simulink model "sf_debouncer_using_duration"  (R2025b)
settings: Solver=VariableStepDiscrete  StartTime=0.0  StopTime=6  RelTol=1e-3  EnableMultiTasking=on
settings Model: Creator=The MathWorks, Inc.  LastModifiedBy=The MathWorks, Inc.
settings SolverCC: AlgebraicLoopSolver=TrustRegion  InsertRTBMode=Auto
settings DataIOCC: LimitDataPoints=on  SaveFormat=Array  ReturnWorkspaceOutputs=off
settings OptimizationCC: ReuseModelBlockBuffer=off  ExpressionDepthLimit=2147483647.0  InitFltsAndDblsToZero=on  EfficientMapNaN2IntZero=off  LifeSpan=inf
settings DebuggingCC: SaveWithParameterizedLinksMsg=none  UnderspecifiedInitializationDetection=Classic  MergeDetectMultiDrivingBlocksExec=none  SignalResolutionControl=TryResolveAllWithWarning  SolverPrmCheckMsg=warning  MultiTaskDSMMsg=warning  MultiTaskCondExecSysMsg=none  FcnCallInpInsideContextMsg=warning  UnconnectedInputMsg=warning  UnconnectedOutputMsg=warning  UnconnectedLineMsg=warning  AllowSymbolicDim=off  StateNameClashWarn=warning  SFUnexpectedBacktrackingDiag=warning  SFNoUnconditionalDefaultTransitionDiag=warning  SFExecutionAtInitializationDiag=none  ArithmeticOperatorsInVariantConditions=warning
settings HardwareCC: ProdBitPerPointer=32.0  ProdBitPerSizeT=32.0  ProdBitPerPtrDiffT=32.0  ProdLargestAtomicFloat=None  ProdIntDivRoundTo=Undefined  ProdEndianess=Unspecified  ProdWordSize=32.0  ProdHWDeviceType=32-bit Generic
settings ModelReferenceCC: EnableRefExpFcnMdlSchedulingChecks=on  PropagateSignalLabelsOutOfModel=off
settings SFSimCC: SimUseLocalCustomCode=off  SimParseCustomCode=off  CustomCodeUndefinedFunction=UseInterfaceOnly
settings RTWCC: RTWUseLocalCustomCode=off  GPUComputeCapability=3.5
settings CodeAppCC: StateflowObjectComments=on
settings GRTTargetCC: TargetFcnLib=ansi_tfl_tmw.mat  TargetLangStandard=C89/C90 (ANSI)  CombineOutputUpdateFcns=off  GRTInterface=on
settings ConfigComp: CovMetricSettings=dw  CovSaveCumulativeToWorkspaceVar=on  CovSaveSingleToWorkspaceVar=on  CovExternalEMLEnable=off  CovSFcnEnable=off

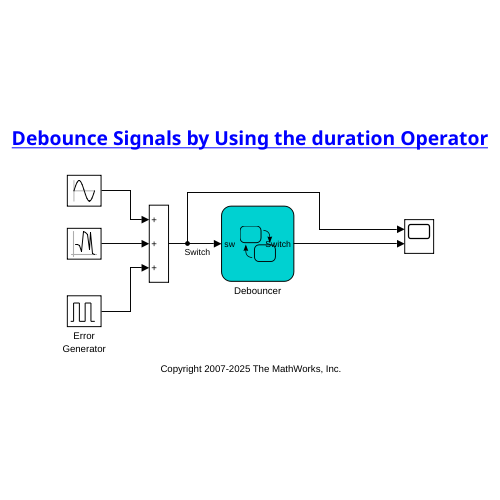
[thumbnail: Simulink's stored preview of the top-level diagram]
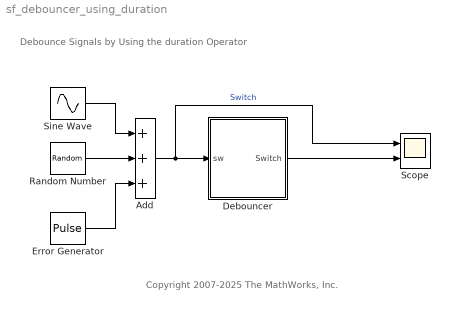
== system sf_debouncer_using_duration ==
  note: Copyright 2007-2025 The MathWorks, Inc.
  note: Debounce Signals by Using the duration Operator
  Add : Sum  Inputs=+++
  Debouncer : Stateflow chart  TreatAsAtomicUnit=on
  Error Generator : DiscretePulseGenerator  PulseType=Time based  Amplitude=10  Period=0.001  PulseWidth=50  PhaseDelay=2
  Random Number : RandomNumber  Variance=30  SampleTime=0
  Scope : Scope  NumInputPorts=2
      settings: TimeSpan=6.5  Title=L_on  ActiveDisplayYMinimum=-44.42228  ActiveDisplayYMaximum=56.97105  DataLoggingMaxPoints=10000
  Sine Wave : Sin  Amplitude=20  Frequency=10  SampleTime=0
  wires:
  Debouncer/1(Switch) -> Scope/2
  Sine Wave/1 -> Add/1
  Random Number/1 -> Add/2
  Add/1 -> Scope/1, Debouncer/1(sw)  "Switch"
  Error Generator/1 -> Add/3

== stateflow chart sf_debouncer_using_duration/Debouncer ==
  settings: updateMethod=DISCRETE  sampleTime=0.001
  state Off
  state On
  (default) -> Off
  On -> Off : [duration(sw < 0) > 0.01]
  Off -> On : [duration(sw >= 0) > 0.01]
  data: sw input; Switch output Enum: SwitchType
